simulink library "ssc_aircraft_elec_lib"  (R2025a)
settings: Solver=VariableStepAuto  StartTime=0.0  StopTime=10.0  RelTol=1e-3
undefined symbols (not defined in the file): Based, FlightProfileChoice, g_norm, Height, payload_mass_workspace, Payload_weight, PowerSystemChoice
libraries: fl_lib x3, aerolibatmos2 x1, nesl_utility x1
Description:
  | Copyright 2017-2025 The MathWorks, Inc.
settings Model: Creator=smiller  LastModifiedBy=smiller
settings SolverCC: AlgebraicLoopSolver=TrustRegion
settings DataIOCC: ReturnWorkspaceOutputs=off
settings OptimizationCC: ReuseModelBlockBuffer=off
settings DebuggingCC: UnconnectedInputMsg=warning  UnconnectedOutputMsg=warning  UnconnectedLineMsg=warning  PregeneratedLibrarySubsystemCodeDiagnostic=none  ArithmeticOperatorsInVariantConditions=warning
settings ModelReferenceCC: EnableRefExpFcnMdlSchedulingChecks=on
settings SFSimCC: SimUseLocalCustomCode=off  CustomCodeUndefinedFunction=UseInterfaceOnly
settings RTWCC: RTWUseLocalCustomCode=off  GPUComputeCapability=3.5  DLArmComputeVersion=19.05
settings CodeAppCC: StateflowObjectComments=on

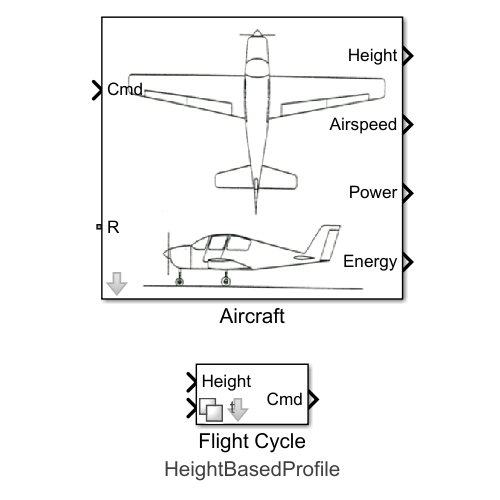
[thumbnail: Simulink's stored preview of the top-level diagram]
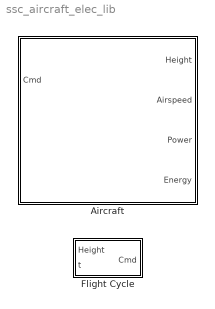
== system ssc_aircraft_elec_lib ==
  Aircraft : Subsystem  mask(Airframe Configuration){popup_aircraft_type=Custom, aircraft_mass_cust=360, aircraft_wing_area_cust=10, aircraft_cl_cust=0.5, aircraft_cd_cust=0.05, aircraft_mass_std=360.000, aircraft_wing_area_std=15.000, aircraft_cl_std=0.055, aircraft_cd_std=0.450, battery_capacity=PowerSystemChoice.battery_capacity, battery_voltage=PowerSystemChoice.battery_voltage, battery_power_density=PowerSystemChoice.power_density, battery_mass=0, engine_system_mass=0, aircraft_max_thrust=PowerSystemChoice.Thrust_max, aircraft_thrust_tau=PowerSystemChoice.tau_T, thrust_eff=0.9, aircraft_h0=FlightProfileChoice.h0, aircraft_v0=0, earth_gravity=g_norm, checkbox_payload_mass=on, payload_mass=Payload_weight}
      mask prompts: popup_aircraft_type "Aircraft Type"; battery_capacity "Capacity (A*hr)"; battery_voltage "Voltage (V)"; battery_power_density "Power Density (W*hr/kg)"; battery_mass "Mass (kg)"; engine_system_mass "Mass Engine System (kg)"; aircraft_max_thrust "Max Thrust (N)"; aircraft_thrust_tau "Thrust Time Constant (s)"; thrust_eff "Thrust Efficiency (0-1)"; aircraft_h0 "Initial Height (m)"; aircraft_v0 "Initial Speed (m/s)"; earth_gravity "Gravity (m/s^2)"; checkbox_payload_mass "Specify Payload Mass in Mask"; payload_mass "Payload Mass (kg)"
      mask help: Define parameters for airframe, including mass, power, and conditions for flight.
      mask init:
      | if(popup_aircraft_type == 1)
      |     aircraft_mass = aircraft_mass_cust;
      |     aircraft_wing_area = aircraft_wing_area_cust;
      |     aircraft_cd = aircraft_cd_cust;
      |     aircraft_cl = aircraft_cl_cust;
      | else
      |     aircraft_mass = aircraft_mass_std;
      |     aircraft_wing_area = aircraft_wing_area_std;
      |     aircraft_cd = aircraft_cd_std;
      |     aircraft_cl = aircraft_cl_std;
      | end
      | 
      | if(checkbox_payload_mass)
      |     use_payload_mass = payload_mass;
      |     set_param([gcb '/Mass/Payload Mass'],'OverrideUsingVariant','Mask');
      | else
      |     use_payload_mass = evalin('base','payload_mass_workspace');
      |     set_param([gcb '/Mass/Payload Mass'],'OverrideUsingVariant','Workspace');
      | end
      | 
      | battery_mass = battery_capacity*battery_voltage/battery_power_density;
      | 
      | total_mass = aircraft_mass+battery_mass+engine_system_mass+use_payload_mass;
      | 
      | [~,~,~,air_rho0] = atmoscoesa(aircraft_h0); 
      | aircraft_v0 = sqrt(2*(total_mass)*earth_gravity/...
      |                             air_rho0/aircraft_cl/aircraft_wing_area);
      mask TypeOptions popup_aircraft_type: Custom | Single Seat Airbus E-Fan | Double Seat Alpha Electro
      mask Callback popup_aircraft_type:
      | maskObj = Simulink.Mask.get(gcb);
      | contca_h = maskObj.getDialogControl('cont_custaircraft');
      | contsa_h = maskObj.getDialogControl('cont_stdaircraft');
      | 
      | airmstd_h = maskObj.getParameter('aircraft_mass_std');
      | airwing_h = maskObj.getParameter('aircraft_wing_area_std');
      | aircd_h = maskObj.getParameter('aircraft_cd_std');
      | aircl_h = maskObj.getParameter('aircraft_cl_std');
      | 
      | popup_at = get_param(gcb,'popup_aircraft_type');
      | if strcmp(popup_at,'Custom')
      |     contca_h.Visible = 'on';
      |     contsa_h.Visible = 'off';
      | else
      |     [temp_mass, temp_area, temp_cd, temp_cl] = ssc_aircraft_elec_props(popup_at);
      |     airmstd_h.ReadOnly = 'off';
      |     airwing_h.ReadOnly = 'off';
      |     aircd_h.ReadOnly = 'off';
      |     aircl_h.ReadOnly = 'off';
      |     set_param(gcb,'aircraft_mass_std',sprintf('%0.3f',temp_mass));
      |     set_param(gcb,'aircraft_wing_area_std',sprintf('%0.3f',temp_area));
      |     set_param(gcb,'aircraft_cd_std',sprintf('%0.3f',temp_cd));
      |     set_param(gcb,'aircraft_cl_std',sprintf('%0.3f',temp_cl));
      | 	airmstd_h.ReadOnly = 'on';
      |     airwing_h.ReadOnly = 'on';
      |     aircd_h.ReadOnly = 'on';
      |     aircl_h.ReadOnly = 'on';
      |     contca_h.Visible = 'off';
      |     contsa_h.Visible = 'on';
      | end
      | 
      | clear maskObj contca_h contsa_h
      | clear airmstd_h airwing_h aircd_h aircl_h
      | clear temp_mass temp_area temp_cd temp_cl
      | clear popup_at
      mask Callback checkbox_payload_mass:
      | maskObj = Simulink.Mask.get(gcb);
      | 
      | payldm_h = maskObj.getParameter('payload_mass');
      | 
      | check_py = get_param(gcb,'checkbox_payload_mass');
      | if (strcmp(check_py,'on'))
      |     payldm_h.Visible = 'on';
      |     set_param([gcb '/Mass/Payload Mass'],'OverrideUsingVariant','Mask');
      | else
      |     payldm_h.Visible = 'off';
      |     set_param([gcb '/Mass/Payload Mass'],'OverrideUsingVariant','Workspace');
      | end
      | 
      | clear maskObj payldm_h
      | clear payldm_h check_py
      mask DialogControl Container6 Prompt: Airframe
      mask DialogControl Control2 Prompt: Aircraft Mass (kg)
      mask DialogControl Control3 Prompt: Wing Equivalent Area (m^2)
      mask DialogControl Control5 Prompt: Coefficient of Lift
      mask DialogControl Control4 Prompt: Coefficient of Drag
      mask DialogControl Container7 Prompt: Power
      mask DialogControl Container13 Prompt: Battery
      mask DialogControl Container8 Prompt: Conditions
      mask Display: image('figuresasbSkyHogg.png');
  Flight Cycle : Subsystem  BlockChoice=Height-Based  Variant=on  mask{popup_flight_cycle_type=Height-Based, flight_cycle_max_height=FlightProfileChoice.FlightProfileHeight, flight_cycle_ascent_start_time=FlightProfileChoice.LevelFlightTime, flight_cycle_duration=FlightProfileChoice.FlightProfileLength, flight_cycle_ascent_duration=FlightProfileChoice.ClimbFlightTime}
      mask prompts: popup_flight_cycle_type "Flight Cycle Type"; flight_cycle_max_height "Maximum Height (m)"; flight_cycle_ascent_start_time "Start time for ascent (sec)"; flight_cycle_duration "Duration of flight cycle (sec)"; flight_cycle_ascent_duration "Duration of ascent (sec)"
      mask init:
      | assignin('base','FlightProfileType',popup_flight_cycle_type);
      settings: AttributesFormatString=%<ActiveVariant>
      mask TypeOptions popup_flight_cycle_type: Height-Based | Time-Based
      mask Display: disp(' ')

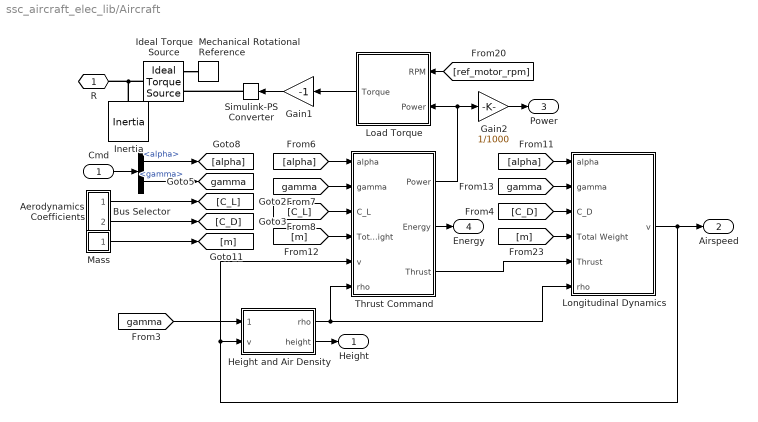
== system ssc_aircraft_elec_lib/Aircraft ==
  Cmd : Inport
  Aerodynamics Coefficients : Subsystem
  Bus Selector : BusSelector  OutputSignals=alpha,gamma
  Gain1 : Gain  Gain=-1
  Gain2 : Gain  Gain=1/1000
  Height and Air Density : Subsystem
  Ideal Torque Source : fl_lib/Mechanical/Mechanical Sources/Ideal Torque Source
  Inertia : fl_lib/Mechanical/Rotational Elements/Inertia  inertia=0.09 kg*m^2  num_ports=foundation.enum.numPorts2.one  w_specify=on  w_priority=High  w=2000 rpm  w_nominal_specify=off  w_nominal_value=1  w_nominal_unit=rad/s  t_specify=off  t_priority=None  t=0 N*m  t_nominal_specify=off  t_nominal_value=1  t_nominal_unit=N*m
  Load Torque : Subsystem  Tag=PublishSubsystem
  Longitudinal Dynamics : Subsystem
  Mass : Subsystem
  Mechanical Rotational Reference : fl_lib/Mechanical/Rotational Elements/Mechanical Rotational Reference
  Simulink-PS Converter : nesl_utility/Simulink-PS Converter  PhysicalDomain=network_engine_domain  SubClassName=ps_input  LeftPortType=input  RightPortType=output  PseudoPeriodic=off  Frequencies=[]  NoiseDistribution=none  NoiseParameters=[]  Unit=1  AffineConversion=off  FilteringAndDerivatives=provide  SimscapeFilterOrder=1  InputFilterTimeConstant=0.001  UdotUserProvided=0
  Thrust Command : Subsystem
  R : PMIOPort  Side=Left
  Height : Outport  VectorParamsAs1DForOutWhenUnconnected=off
  Airspeed : Outport  Port=2  VectorParamsAs1DForOutWhenUnconnected=off
  Power : Outport  Port=3  VectorParamsAs1DForOutWhenUnconnected=off
  Energy : Outport  Port=4  VectorParamsAs1DForOutWhenUnconnected=off
  tag scope: gamma=global
  wires:
  [gamma] -> Thrust Command/2(gamma)
  [C_L] -> Thrust Command/3(C_L)
  [C_D] -> Longitudinal Dynamics/3(C_D)
  Height and Air Density/1(rho) -> Longitudinal Dynamics/6(rho), Thrust Command/6(rho)
  [gamma] -> Longitudinal Dynamics/2(gamma)
  Aerodynamics Coefficients/2(cd) -> [C_D]
  [gamma] -> Height and Air Density/1(gamma)
  Aerodynamics Coefficients/1(cl) -> [C_L]
  [alpha] -> Longitudinal Dynamics/1(alpha)
  [alpha] -> Thrust Command/1(alpha)
  Longitudinal Dynamics/1(v) -> Airspeed/1, Height and Air Density/2(v), Thrust Command/5(v)
  Thrust Command/3(Thrust) -> Longitudinal Dynamics/5(Thrust)
  Thrust Command/1(Power) -> Gain2/1, Load Torque/2(Power)
  Height and Air Density/2(height) -> Height/1
  Gain1/1 -> Simulink-PS Converter/1
  [ref_motor_rpm] -> Load Torque/1(RPM)
  Load Torque/1(Torque) -> Gain1/1
  Gain2/1 -> Power/1
  Thrust Command/2(Energy) -> Energy/1
  Bus Selector/2 -> [gamma]  "<gamma>"
  Cmd/1 -> Bus Selector/1
  Bus Selector/1 -> [alpha]  "<alpha>"
  Mass/1(m) -> [m]
  [m] -> Longitudinal Dynamics/4(Total Weight)
  [m] -> Thrust Command/4(Total Weight)
  connections:
  Simulink-PS Converter/RConn1 -- Ideal Torque Source/RConn1
  Ideal Torque Source/LConn1 -- R/RConn1 -- Inertia/LConn1
  Ideal Torque Source/RConn2 -- Mechanical Rotational Reference/LConn1

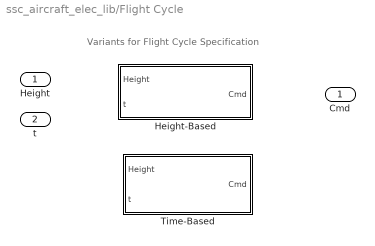
== system ssc_aircraft_elec_lib/Flight Cycle ==
  note: Variants for Flight Cycle Specification
  Height : Inport
  "      t" : Inport  Port=2
  Height-Based : Subsystem  VariantControl=HeightBasedProfile  mask{cycle_max_height=flight_cycle_max_height, cycle_max_length=flight_cycle_duration, time_start_ascent=flight_cycle_ascent_start_time}
      mask prompts: cycle_max_height "Maximum Height (m)"; cycle_max_length "Maximum Length (m)"; time_start_ascent "Start time for ascent (sec)"
  Time-Based : Subsystem  VariantControl=TimeBasedProfile  mask{time_ascent_start=flight_cycle_ascent_start_time, time_ascent_duration=flight_cycle_ascent_duration, time_cycle_duration=flight_cycle_duration}
      mask prompts: time_ascent_start "Start time for ascent (sec)"; time_ascent_duration "Duration of ascent (sec)"; time_cycle_duration "Duration of flight cycle (sec)"
  Cmd : Outport  VectorParamsAs1DForOutWhenUnconnected=off

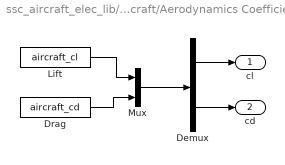
== system ssc_aircraft_elec_lib/Aircraft/Aerodynamics Coefficients ==
  Demux : Demux  Outputs=2
  Drag : Constant  Value=aircraft_cd
  Lift : Constant  Value=aircraft_cl
  Mux : Mux  Inputs=2
  cl : Outport  VectorParamsAs1DForOutWhenUnconnected=off
  cd : Outport  Port=2  VectorParamsAs1DForOutWhenUnconnected=off
  wires:
  Demux/1 -> cl/1
  Demux/2 -> cd/1
  Lift/1 -> Mux/1
  Drag/1 -> Mux/2
  Mux/1 -> Demux/1

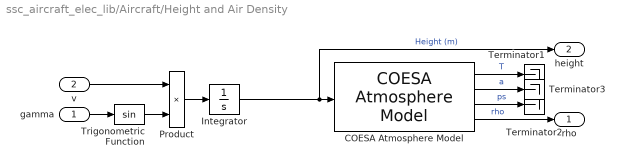
== system ssc_aircraft_elec_lib/Aircraft/Height and Air Density ==
  gamma : Inport
  v : Inport  Port=2
  COESA Atmosphere Model : aerolibatmos2/COESA Atmosphere Model  units=Metric (MKS)  spec=1976 COESA-extended U.S. Standard Atmosphere  model=Profile  profile_var=High temperature  profile_percent=1%  profile_alt=5 km (16404 ft)  envelope_var=High temperature  envelope_percent=1%  action=Warning
  Integrator : Integrator  InitialCondition=aircraft_h0
  Product : Product
  Terminator1 : Terminator
  Terminator2 : Terminator
  Terminator3 : Terminator
  Trigonometric Function : Trigonometry
  rho : Outport  VectorParamsAs1DForOutWhenUnconnected=off
  height : Outport  Port=2  VectorParamsAs1DForOutWhenUnconnected=off
  wires:
  COESA Atmosphere Model/4 -> rho/1  "rho"
  Trigonometric Function/1 -> Product/2
  Integrator/1 -> height/1, COESA Atmosphere Model/1  "Height (m)"
  COESA Atmosphere Model/3 -> Terminator2/1  "ps"
  COESA Atmosphere Model/2 -> Terminator3/1  "a"
  COESA Atmosphere Model/1 -> Terminator1/1  "T"
  Product/1 -> Integrator/1
  v/1 -> Product/1
  gamma/1 -> Trigonometric Function/1

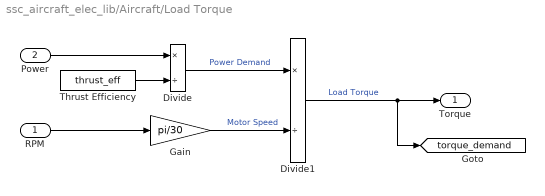
== system ssc_aircraft_elec_lib/Aircraft/Load Torque ==
  RPM : Inport
  Power : Inport  Port=2
  Divide : Product  Inputs=*/
  Divide1 : Product  Inputs=*/
  Gain : Gain  Gain=pi/30
  Thrust Efficiency : Constant  Value=thrust_eff
  Torque : Outport  VectorParamsAs1DForOutWhenUnconnected=off
  tag scope: torque_demand=global
  wires:
  Thrust Efficiency/1 -> Divide/2
  Power/1 -> Divide/1
  Divide/1 -> Divide1/1  "Power Demand"
  Divide1/1 -> Torque/1, [torque_demand]  "Load Torque"
  Gain/1 -> Divide1/2  "Motor Speed"
  RPM/1 -> Gain/1

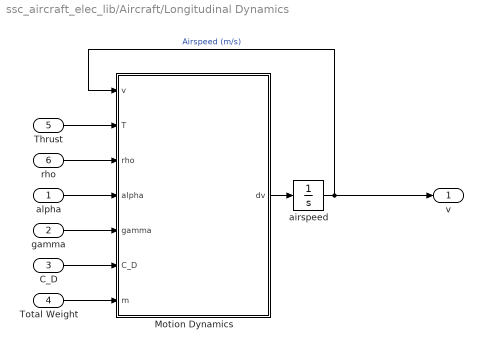
== system ssc_aircraft_elec_lib/Aircraft/Longitudinal Dynamics ==
  alpha : Inport
  gamma : Inport  Port=2
  C_D : Inport  Port=3
  Total Weight : Inport  Port=4
  Thrust : Inport  Port=5
  rho : Inport  Port=6
  Motion Dynamics : MATLAB Function  TreatAsAtomicUnit=on  mask{Sw=aircraft_wing_area, g=g_norm}
      mask prompts: Sw "Equivalent Area (m^2)"; g "Gravity Constant"
  airspeed : Integrator  InitialCondition=aircraft_v0
  v : Outport  VectorParamsAs1DForOutWhenUnconnected=off
  wires:
  Thrust/1 -> Motion Dynamics/2(T)
  rho/1 -> Motion Dynamics/3(rho)
  gamma/1 -> Motion Dynamics/5(gamma)
  alpha/1 -> Motion Dynamics/4(alpha)
  C_D/1 -> Motion Dynamics/6(C_D)
  Motion Dynamics/1(dv) -> airspeed/1
  airspeed/1 -> Motion Dynamics/1(v), v/1  "Airspeed (m/s)"
  Total Weight/1 -> Motion Dynamics/7(m)

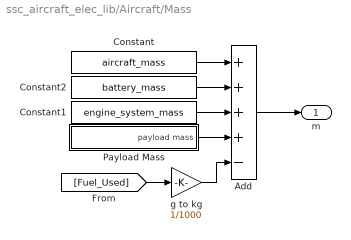
== system ssc_aircraft_elec_lib/Aircraft/Mass ==
  Add : Sum  Inputs=++++-
  Constant : Constant  Value=aircraft_mass
  Constant1 : Constant  Value=engine_system_mass
  Constant2 : Constant  Value=battery_mass
  Payload Mass : Subsystem  Variant=on  VariantControlMode=label  VariantControl=Variant1  LabelModeActiveChoice=Mask
  g to kg : Gain  Gain=1/1000
  m : Outport  VectorParamsAs1DForOutWhenUnconnected=off
  wires:
  Constant/1 -> Add/1
  Add/1 -> m/1
  [Fuel_Used] -> g to kg/1
  g to kg/1 -> Add/5
  Constant2/1 -> Add/2
  Payload Mass/1(" payload mass") -> Add/4
  Constant1/1 -> Add/3

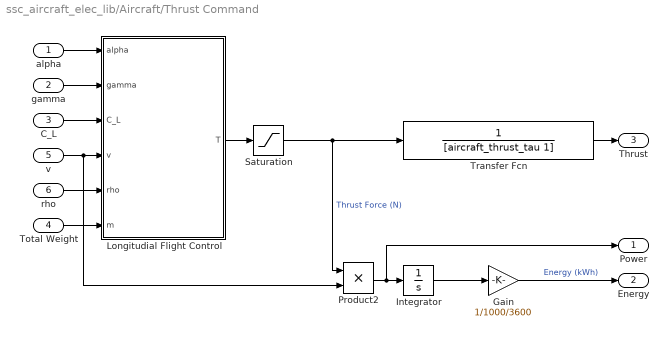
== system ssc_aircraft_elec_lib/Aircraft/Thrust Command ==
  alpha : Inport
  gamma : Inport  Port=2
  C_L : Inport  Port=3
  Total Weight : Inport  Port=4
  v : Inport  Port=5
  rho : Inport  Port=6
  Gain : Gain  Gain=1/1000/3600
  Integrator : Integrator
  Longitudial Flight Control : MATLAB Function  TreatAsAtomicUnit=on  mask{Sw=aircraft_wing_area, g=g_norm}
      mask prompts: Sw "Equivalent Area (m^2)"; g "Gravity Constant"
  Product2 : Product
  Saturation : Saturate  UpperLimit=aircraft_max_thrust  LowerLimit=0
  Transfer Fcn : TransferFcn  Denominator=[aircraft_thrust_tau 1]
  Power : Outport  VectorParamsAs1DForOutWhenUnconnected=off
  Energy : Outport  Port=2  VectorParamsAs1DForOutWhenUnconnected=off
  Thrust : Outport  Port=3  VectorParamsAs1DForOutWhenUnconnected=off
  wires:
  alpha/1 -> Longitudial Flight Control/1(alpha)
  rho/1 -> Longitudial Flight Control/5(rho)
  v/1 -> Product2/2, Longitudial Flight Control/4(v)
  Transfer Fcn/1 -> Thrust/1
  Longitudial Flight Control/1(T) -> Saturation/1
  Saturation/1 -> Transfer Fcn/1, Product2/1  "Thrust Force (N)"
  Product2/1 -> Power/1, Integrator/1
  Integrator/1 -> Gain/1
  Gain/1 -> Energy/1  "Energy (kWh)"
  C_L/1 -> Longitudial Flight Control/3(C_L)
  gamma/1 -> Longitudial Flight Control/2(gamma)
  Total Weight/1 -> Longitudial Flight Control/6(m)

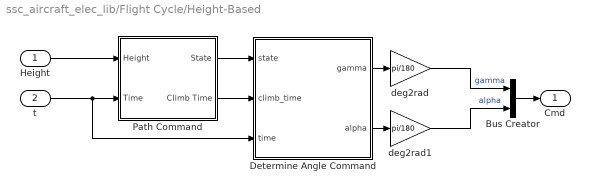
== system ssc_aircraft_elec_lib/Flight Cycle/Height-Based ==
  Height : Inport
  "    t" : Inport  Port=2
  Bus Creator : BusCreator  Inputs=2
  Determine Angle Command : MATLAB Function  TreatAsAtomicUnit=on  mask{timeMax=cycle_max_length}
      mask prompts: timeMax "Maximum Length of Flight Profile"
  Path Command : Subsystem
  deg2rad : Gain  Gain=pi/180
  deg2rad1 : Gain  Gain=pi/180
  Cmd : Outport  VectorParamsAs1DForOutWhenUnconnected=off
  wires:
  deg2rad1/1 -> Bus Creator/2  "alpha"
  Bus Creator/1 -> Cmd/1
  Determine Angle Command/1(gamma) -> deg2rad/1
  Determine Angle Command/2(alpha) -> deg2rad1/1
  Path Command/1(State) -> Determine Angle Command/1(state)
  Path Command/2(Climb Time) -> Determine Angle Command/2(climb_time)
  deg2rad/1 -> Bus Creator/1  "gamma"
  "    t"/1 -> Path Command/2(Time), Determine Angle Command/3(time)
  Height/1 -> Path Command/1(Height)

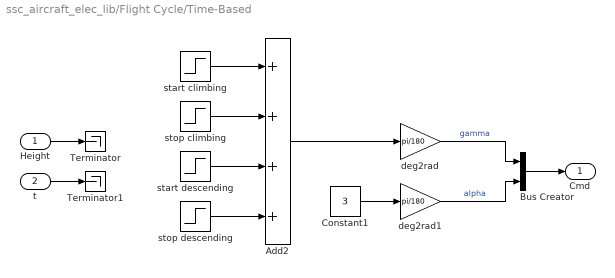
== system ssc_aircraft_elec_lib/Flight Cycle/Time-Based ==
  Height : Inport
  "    t" : Inport  Port=2
  Add2 : Sum  Inputs=++++
  Bus Creator : BusCreator  Inputs=2
  Constant1 : Constant  Value=3
  Terminator : Terminator
  Terminator1 : Terminator
  deg2rad : Gain  Gain=pi/180
  deg2rad1 : Gain  Gain=pi/180
  start climbing : Step  Time=time_ascent_start  SampleTime=0
  start descending : Step  Time=time_cycle_duration - time_ascent_duration - time_ascent_start  After=-1  SampleTime=0
  stop climbing : Step  Time=time_ascent_start+time_ascent_duration  After=-1  SampleTime=0
  stop descending : Step  Time=time_cycle_duration - time_ascent_start  SampleTime=0
  Cmd : Outport  VectorParamsAs1DForOutWhenUnconnected=off
  wires:
  Constant1/1 -> deg2rad1/1
  Add2/1 -> deg2rad/1
  stop climbing/1 -> Add2/2
  deg2rad/1 -> Bus Creator/1  "gamma"
  start climbing/1 -> Add2/1
  start descending/1 -> Add2/3
  stop descending/1 -> Add2/4
  Bus Creator/1 -> Cmd/1
  deg2rad1/1 -> Bus Creator/2  "alpha"
  Height/1 -> Terminator/1
  "    t"/1 -> Terminator1/1

== system ssc_aircraft_elec_lib/Aircraft/Mass/Payload Mass ==
  Mask : Subsystem  VariantControl=Mask
  Workspace : Subsystem  VariantControl=Workspace
  " payload mass" : Outport  VectorParamsAs1DForOutWhenUnconnected=off

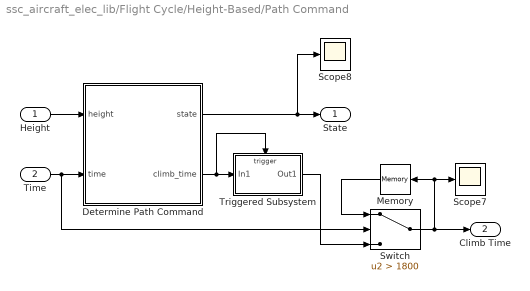
== system ssc_aircraft_elec_lib/Flight Cycle/Height-Based/Path Command ==
  Height : Inport
  Time : Inport  Port=2
  Determine Path Command : MATLAB Function  TreatAsAtomicUnit=on  mask{heightMax=cycle_max_height, timeMax=cycle_max_length, timeLevel=time_start_ascent}
      mask prompts: heightMax "Maximum Height of Flight Profile"; timeMax "Maximum Length of Flight Profile"; timeLevel "Level Flight Time"
  Memory : Memory
  Scope7 : Scope
      settings: ActiveDisplayYMinimum=-139.82678  ActiveDisplayYMaximum=1258.44098  DataLoggingVariableName=ScopeData3
  Scope8 : Scope
      settings: ActiveDisplayYMinimum=-0.125  ActiveDisplayYMaximum=1.125  DataLoggingVariableName=ScopeData4
  Switch : Switch  Criteria=u2 > Threshold  Threshold=1800  SaturateOnIntegerOverflow=off  InputSameDT=off
  Triggered Subsystem : Subsystem  TreatAsAtomicUnit=on
  State : Outport  VectorParamsAs1DForOutWhenUnconnected=off
  Climb Time : Outport  Port=2  VectorParamsAs1DForOutWhenUnconnected=off
  wires:
  Triggered Subsystem/1(Out1) -> Switch/3
  Switch/1 -> Climb Time/1, Memory/1, Scope7/1
  Determine Path Command/2(climb_time) -> Triggered Subsystem/1(In1), Triggered Subsystem/Trigger
  Determine Path Command/1(state) -> Scope8/1, State/1
  Memory/1 -> Switch/1
  Time/1 -> Determine Path Command/2(time), Switch/2
  Height/1 -> Determine Path Command/1(height)

== system ssc_aircraft_elec_lib/Aircraft/Mass/Payload Mass/Mask ==
  Payload Mass : Constant  Value=payload_mass
  payload mass : Outport  VectorParamsAs1DForOutWhenUnconnected=off
  wires:
  Payload Mass/1 -> payload mass/1

== system ssc_aircraft_elec_lib/Aircraft/Mass/Payload Mass/Workspace ==
  Payload Mass1 : Constant  Value=payload_mass_workspace
  " payload mass" : Outport  VectorParamsAs1DForOutWhenUnconnected=off
  wires:
  Payload Mass1/1 -> " payload mass"/1

== system ssc_aircraft_elec_lib/Flight Cycle/Height-Based/Path Command/Triggered Subsystem ==
  In1 : Inport
  Trigger : TriggerPort  VariantControl=Variant
  Out1 : Outport  VectorParamsAs1DForOutWhenUnconnected=off
  wires:
  In1/1 -> Out1/1

== matlab function ssc_aircraft_elec_lib/Aircraft/Thrust Command/Longitudial Flight Control ==
  data: alpha input; gamma input; C_L input; T output; g parameter; v input; rho input; Sw parameter; m input
function T  = longFlightControl(alpha, gamma, C_L, g, v, rho, Sw, m)

T = 1/sin(alpha)*(m*g*cos(gamma)-1/2*rho*v^2*C_L*Sw);

== matlab function ssc_aircraft_elec_lib/Aircraft/Longitudinal Dynamics/Motion Dynamics ==
  data: v input; dv output; T input; rho input; alpha input; gamma input; Sw parameter; g parameter; C_D input; m input
function dv  = motionDynamics(v, T, rho, alpha, gamma, Sw, g, C_D, m)

dv = -1/2*rho*v^2*C_D*Sw/m - g*sin(gamma) + T*cos(alpha)/m;

== matlab function ssc_aircraft_elec_lib/Flight Cycle/Height-Based/Determine Angle Command ==
  data: gamma output; state input; climb_time input; alpha output; time input; timeMax parameter
function [gamma, alpha] = angleCommand(state, climb_time, time, timeMax)

if state == 2
    gamma = 0;
    alpha = 3;
else
    if state == 0
        gamma = 1;
        alpha = 3;
    else
        if time < (timeMax - climb_time)
        gamma = 0;
        alpha = 3;
        else
        gamma = -1;
        alpha = 3; 
        end
    end
end

== matlab function ssc_aircraft_elec_lib/Flight Cycle/Height-Based/Path Command/Determine Path Command ==
  data: state output; height input; climb_time output; time input; heightMax parameter; timeMax parameter; timeLevel parameter
function [state, climb_time] = pathCommand(height, time, heightMax, timeMax, timeLevel)
climb_time = 0;
state = 0;

if time < timeLevel
    state = 2;
else    
    if height < heightMax && time < timeMax/2
        state = 0;
    else
        if climb_time == 0
            climb_time = time-timeLevel;
        end
        state = 1;
    end
end
